simulink model "cov_compare"  (Simulink 5.0)
settings: Solver=ode45  StartTime=0.0  StopTime=10.0  RelTol=1e-3
values from neighbouring files (symbols this model uses):
  I = eye(3)    [build17StateSysDyn.m]    (also in build9StateSysDyn.m; cmigits28_model_01.mat = [1 0 0 0 0 0 0 0 0 0 0 0 ... (784 elements, 28x28)]; covupdate.m = eye(m))
undefined symbols (not defined in the file or in its folder): F1, F2, H1, H2, P1_0, P2_0, Q1, Q2, R1, R2, rss_ratio, ud_inv
libraries: simulink x4
settings Model: Creator=mcarroll  LastModifiedBy=mcarroll  ExtModeAutoUpdateStatusClock=off  SaveFormat=StructureWithTime

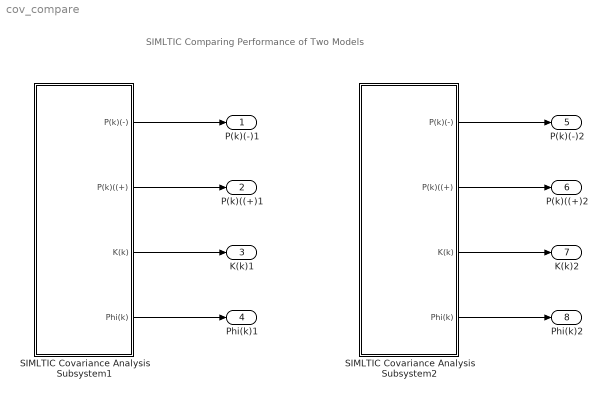
== system cov_compare ==
  note: SIMLTIC
      | Comparing Performance of Two Models
  SIMLTIC Covariance Analysis Subsystem1 : Subsystem
  SIMLTIC Covariance Analysis Subsystem2 : Subsystem
  P(k)(-)1 : Outport
  P(k)((+)1 : Outport  Port=2
  K(k)1 : Outport  Port=3
  Phi(k)1 : Outport  Port=4
  P(k)(-)2 : Outport  Port=5
  P(k)((+)2 : Outport  Port=6
  K(k)2 : Outport  Port=7
  Phi(k)2 : Outport  Port=8
  wires:
  SIMLTIC Covariance Analysis Subsystem1/1(P(k)(-)) -> P(k)(-)1/1
  SIMLTIC Covariance Analysis Subsystem1/2(P(k)((+)) -> P(k)((+)1/1
  SIMLTIC Covariance Analysis Subsystem1/3(K(k)) -> K(k)1/1
  SIMLTIC Covariance Analysis Subsystem1/4(Phi(k)) -> Phi(k)1/1
  SIMLTIC Covariance Analysis Subsystem2/1(P(k)(-)) -> P(k)(-)2/1
  SIMLTIC Covariance Analysis Subsystem2/2(P(k)((+)) -> P(k)((+)2/1
  SIMLTIC Covariance Analysis Subsystem2/3(K(k)) -> K(k)2/1
  SIMLTIC Covariance Analysis Subsystem2/4(Phi(k)) -> Phi(k)2/1

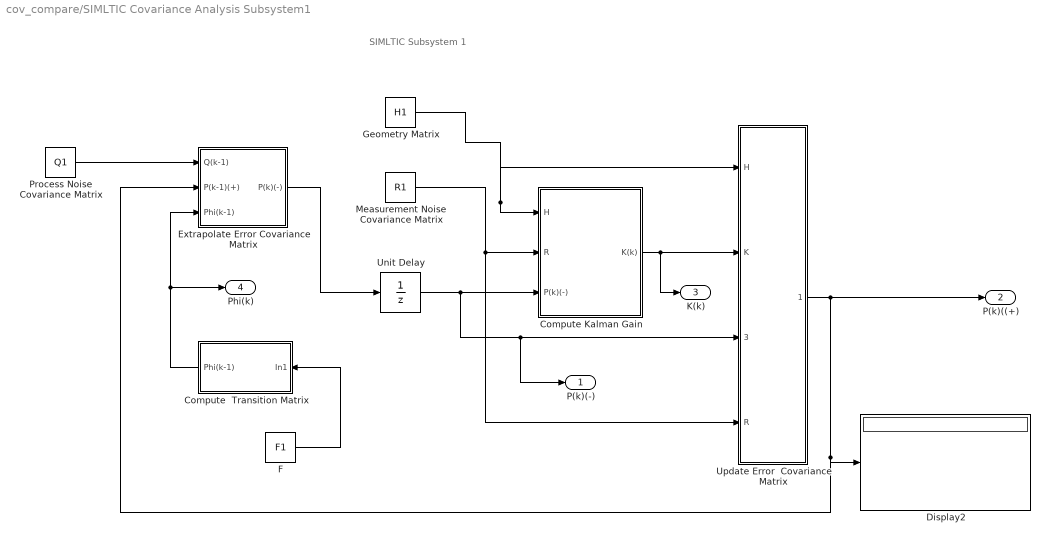
== system cov_compare/SIMLTIC Covariance Analysis Subsystem1 ==
  note: SIMLTIC
      | Subsystem 1
  Compute  Transition Matrix : Subsystem  Orientation=left
  Compute Kalman Gain : Subsystem
  Display2 : Display
  Extrapolate Error Covariance Matrix : Subsystem
  F : Constant  Value=F1  VectorParams1D=off
  Geometry Matrix : Constant  Value=H1  VectorParams1D=off
  Measurement Noise Covariance Matrix : Constant  Value=R1  VectorParams1D=off
  Process Noise Covariance Matrix : Constant  Value=Q1  VectorParams1D=off
  Unit Delay : UnitDelay  X0=P1_0
  Update Error  Covariance Matrix : Subsystem
  P(k)(-) : Outport
  P(k)((+) : Outport  Port=2
  K(k) : Outport  Port=3
  Phi(k) : Outport  Port=4
  wires:
  F/1 -> Compute  Transition Matrix/1(In1)
  Measurement Noise Covariance Matrix/1 -> Update Error  Covariance Matrix/4(R), Compute Kalman Gain/2(R)
  Geometry Matrix/1 -> Update Error  Covariance Matrix/1(H), Compute Kalman Gain/1(H)
  Compute  Transition Matrix/1(Phi(k-1)) -> Phi(k)/1, Extrapolate Error Covariance Matrix/3(Phi(k-1))
  Extrapolate Error Covariance Matrix/1(P(k)(-)) -> Unit Delay/1
  Process Noise Covariance Matrix/1 -> Extrapolate Error Covariance Matrix/1(Q(k-1))
  Compute Kalman Gain/1(K(k)) -> K(k)/1, Update Error  Covariance Matrix/2(K)
  Unit Delay/1 -> P(k)(-)/1, Update Error  Covariance Matrix/3(P(k)(-)), Compute Kalman Gain/3(P(k)(-))
  Update Error  Covariance Matrix/1(P(k)(+)) -> P(k)((+)/1, Extrapolate Error Covariance Matrix/2(P(k-1)(+)), Display2/1

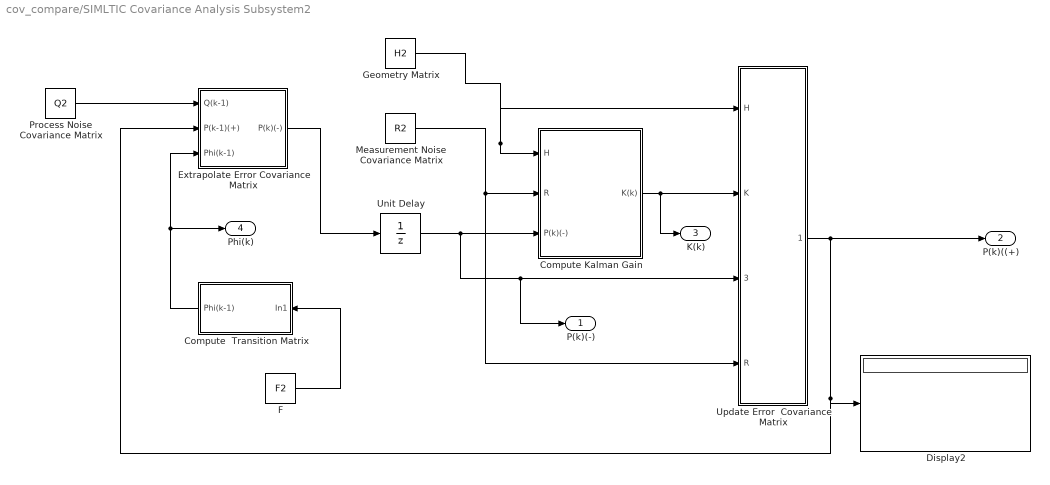
== system cov_compare/SIMLTIC Covariance Analysis Subsystem2 ==
  Compute  Transition Matrix : Subsystem  Orientation=left
  Compute Kalman Gain : Subsystem
  Display2 : Display
  Extrapolate Error Covariance Matrix : Subsystem
  F : Constant  Value=F2  VectorParams1D=off
  Geometry Matrix : Constant  Value=H2  VectorParams1D=off
  Measurement Noise Covariance Matrix : Constant  Value=R2  VectorParams1D=off
  Process Noise Covariance Matrix : Constant  Value=Q2  VectorParams1D=off
  Unit Delay : UnitDelay  X0=P2_0
  Update Error  Covariance Matrix : Subsystem
  P(k)(-) : Outport
  P(k)((+) : Outport  Port=2
  K(k) : Outport  Port=3
  Phi(k) : Outport  Port=4
  wires:
  Update Error  Covariance Matrix/1(P(k)(+)) -> Display2/1, Extrapolate Error Covariance Matrix/2(P(k-1)(+)), P(k)((+)/1
  Unit Delay/1 -> Compute Kalman Gain/3(P(k)(-)), Update Error  Covariance Matrix/3(P(k)(-)), P(k)(-)/1
  Compute Kalman Gain/1(K(k)) -> Update Error  Covariance Matrix/2(K), K(k)/1
  Process Noise Covariance Matrix/1 -> Extrapolate Error Covariance Matrix/1(Q(k-1))
  Extrapolate Error Covariance Matrix/1(P(k)(-)) -> Unit Delay/1
  Compute  Transition Matrix/1(Phi(k-1)) -> Extrapolate Error Covariance Matrix/3(Phi(k-1)), Phi(k)/1
  Geometry Matrix/1 -> Compute Kalman Gain/1(H), Update Error  Covariance Matrix/1(H)
  Measurement Noise Covariance Matrix/1 -> Compute Kalman Gain/2(R), Update Error  Covariance Matrix/4(R)
  F/1 -> Compute  Transition Matrix/1(In1)

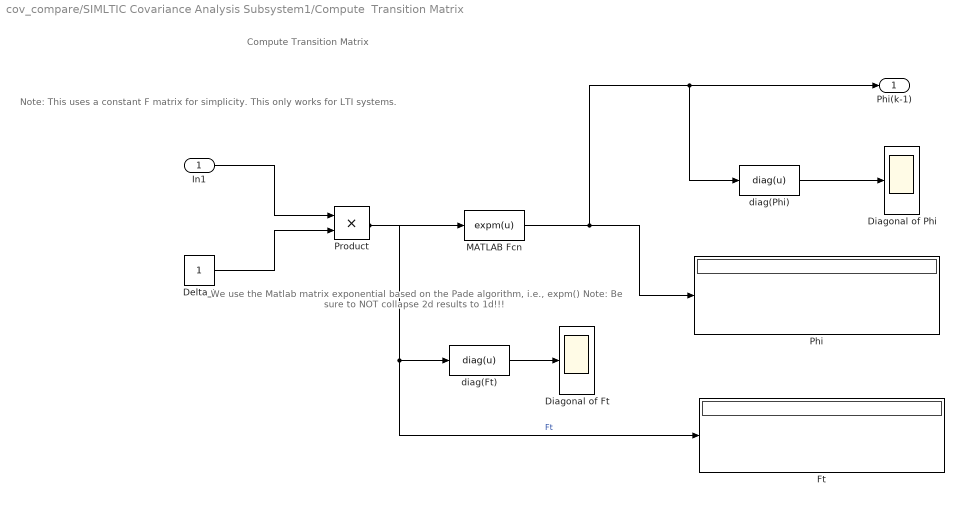
== system cov_compare/SIMLTIC Covariance Analysis Subsystem1/Compute  Transition Matrix ==
  note: Compute Transition Matrix
  note: Note:  This uses a constant F matrix
      | for simplicity.  This only works for LTI
      | systems.
  note: We use the Matlab matrix exponential based
      | on the Pade algorithm, i.e., expm()
      | Note:  Be sure to NOT collapse 2d results
      | to 1d!!!
  In1 : Inport
  Delta_t : Constant
  Diagonal of Ft : Scope
      settings: YMin=0  YMax=2  SaveName=ScopeData18
  Diagonal of Phi : Scope
      settings: YMin=0  YMax=2  SaveName=ScopeData3
  Ft : Display
  MATLAB Fcn : MATLABFcn  MATLABFcn=expm(u)  Output1D=off
  Phi : Display
  Product : Product  SaturateOnIntegerOverflow=on  InputSameDT=on
  diag(Ft) : MATLABFcn  MATLABFcn=diag(u)  Output1D=off
  diag(Phi) : MATLABFcn  MATLABFcn=diag(u)
  Phi(k-1) : Outport
  wires:
  In1/1 -> Product/1
  Product/1 -> MATLAB Fcn/1, Ft/1, diag(Ft)/1  "Ft"
  MATLAB Fcn/1 -> Phi/1, Phi(k-1)/1, diag(Phi)/1
  diag(Phi)/1 -> Diagonal of Phi/1
  diag(Ft)/1 -> Diagonal of Ft/1
  Delta_t/1 -> Product/2

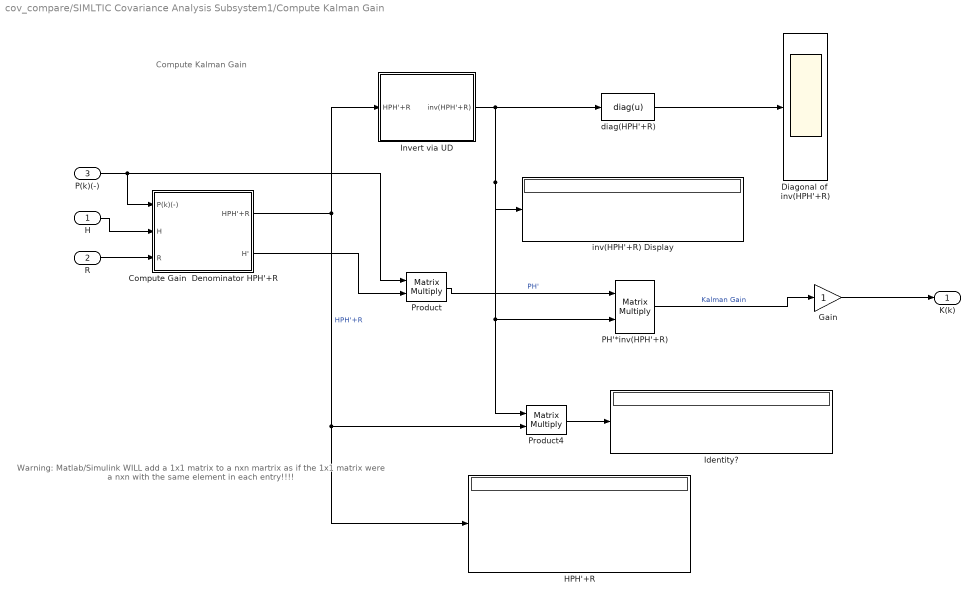
== system cov_compare/SIMLTIC Covariance Analysis Subsystem1/Compute Kalman Gain ==
  note: Warning:
      | Matlab/Simulink
      | WILL add a 1x1 matrix to
      | a nxn martrix as if the
      | 1x1 matrix were a
      | nxn with the same element
      | in each entry!!!!
  note: Compute Kalman Gain
  H : Inport
  R : Inport  Port=2
  P(k)(-) : Inport  Port=3  ShowAdditionalParam=on
  Compute Gain  Denominator HPH'+R : Subsystem
  Diagonal of  inv(HPH'+R) : Scope
      settings: TimeRange=100  YMin=0.0006  YMax=0.002  SaveName=ScopeData2
  Gain : Gain  SaturateOnIntegerOverflow=on
  HPH'+R : Display
  Identity? : Display
  Invert via UD : Subsystem
  PH'*inv(HPH'+R) : Product  Multiplication=Matrix(*)  ShowAdditionalParam=on
  Product : Product  Multiplication=Matrix(*)  SaturateOnIntegerOverflow=on
  Product4 : Product  Multiplication=Matrix(*)  ShowAdditionalParam=on  SaturateOnIntegerOverflow=on  InputSameDT=on
  diag(HPH'+R) : MATLABFcn  MATLABFcn=diag(u)
  inv(HPH'+R) Display : Display
  K(k) : Outport
  wires:
  Gain/1 -> K(k)/1
  PH'*inv(HPH'+R)/1 -> Gain/1  "Kalman Gain"
  P(k)(-)/1 -> Product/1, Compute Gain  Denominator HPH'+R/1(P(k)(-))
  H/1 -> Compute Gain  Denominator HPH'+R/2(H)
  Product4/1 -> Identity?/1
  Product/1 -> PH'*inv(HPH'+R)/1  "PH'"
  Compute Gain  Denominator HPH'+R/2(H') -> Product/2
  Invert via UD/1(inv(HPH'+R)) -> Product4/1, PH'*inv(HPH'+R)/2, inv(HPH'+R) Display/1, diag(HPH'+R)/1
  diag(HPH'+R)/1 -> Diagonal of  inv(HPH'+R)/1
  R/1 -> Compute Gain  Denominator HPH'+R/3(R)
  Compute Gain  Denominator HPH'+R/1(HPH'+R) -> Product4/2, HPH'+R/1, Invert via UD/1(HPH'+R)  "HPH'+R"

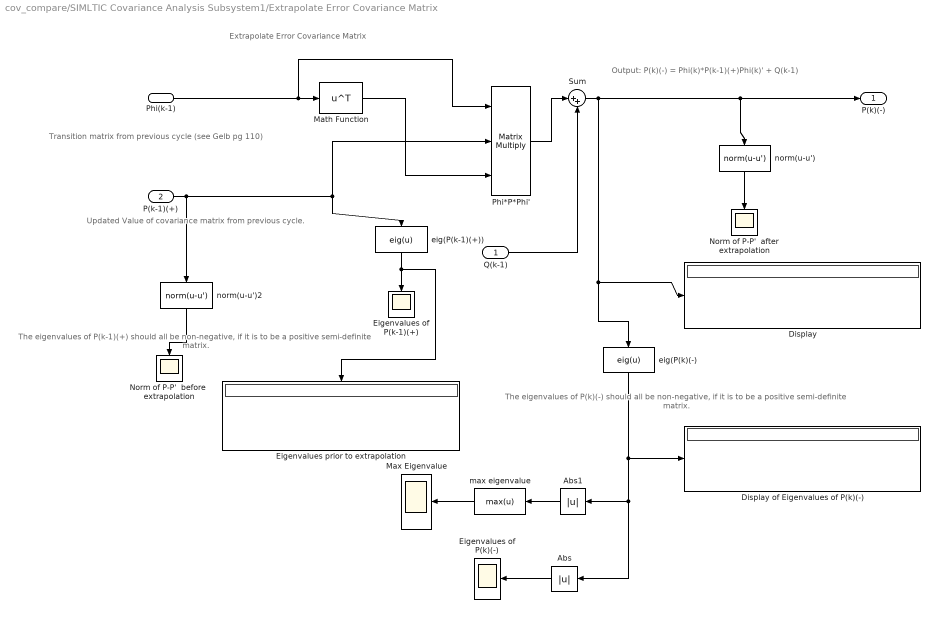
== system cov_compare/SIMLTIC Covariance Analysis Subsystem1/Extrapolate Error Covariance Matrix ==
  note: Extrapolate Error Covariance Matrix
  note: Updated Value of
      | covariance matrix  from
      | previous cycle.
  note: Output: P(k)(-) = Phi(k)*P(k-1)(+)Phi(k)' + Q(k-1)
  note: Transition matrix from
      | previous cycle
      | (see Gelb pg 110)
  note: The eigenvalues of P(k-1)(+) should all be
      | non-negative, if it is to be a positive
      | semi-definite matrix.
  note: The eigenvalues of P(k)(-) should all be non-negative,
      | if it is to be a positive semi-definite matrix.
  Q(k-1) : Inport
  P(k-1)(+) : Inport  Port=2
  Phi(k-1) : Inport  Port=3
  Abs : Abs  Orientation=left  SaturateOnIntegerOverflow=on
  Abs1 : Abs  Orientation=left  SaturateOnIntegerOverflow=on
  Display : Display
  Display of Eigenvalues of P(k)(-) : Display
  Eigenvalues prior to extrapolation : Display
      settings: Orientation=down
  Eigenvalues of P(k)(-) : Scope
      settings: SaveName=ScopeData8
  Eigenvalues of P(k-1)(+) : Scope
      settings: Orientation=down  YMin=1  YMax=8.5  SaveName=ScopeData7
  Math Function : Math  Operator=transpose
  Max Eigenvalue : Scope
      settings: TimeRange=100  YMin=0  YMax=4e+072  SaveName=ScopeData12
  Norm of P-P'  after extrapolation : Scope
      settings: Orientation=down  TimeRange=10  YMin=0  YMax=35  SaveName=ScopeData15
  Norm of P-P'  before  extrapolation : Scope
      settings: Orientation=down  TimeRange=10  YMin=0  YMax=35  SaveName=ScopeData16
  Phi*P*Phi' : Product  Inputs=3  Multiplication=Matrix(*)  SaturateOnIntegerOverflow=on  InputSameDT=on
  Sum : Sum  Inputs=|++  SaturateOnIntegerOverflow=on  InputSameDT=on
  eig(P(k)(-) : MATLABFcn  Orientation=down  MATLABFcn=eig(u)  OutputSignalType=complex
  eig(P(k-1)(+)) : MATLABFcn  Orientation=down  MATLABFcn=eig(u)
  max eigenvalue : MATLABFcn  Orientation=left  MATLABFcn=max(u)  Output1D=off
  norm(u-u') : MATLABFcn  Orientation=down  MATLABFcn=norm(u-u')  Output1D=off
  norm(u-u')2 : MATLABFcn  Orientation=down  MATLABFcn=norm(u-u')  Output1D=off
  P(k)(-) : Outport
  wires:
  Phi*P*Phi'/1 -> Sum/1
  Sum/1 -> Display/1, eig(P(k)(-)/1, P(k)(-)/1, norm(u-u')/1
  Phi(k-1)/1 -> Math Function/1, Phi*P*Phi'/1
  P(k-1)(+)/1 -> norm(u-u')2/1, eig(P(k-1)(+))/1, Phi*P*Phi'/2
  Q(k-1)/1 -> Sum/2
  eig(P(k-1)(+))/1 -> Eigenvalues of P(k-1)(+)/1, Eigenvalues prior to extrapolation/1
  eig(P(k)(-)/1 -> Display of Eigenvalues of P(k)(-)/1, Abs/1, Abs1/1
  norm(u-u')/1 -> Norm of P-P'  after extrapolation/1
  norm(u-u')2/1 -> Norm of P-P'  before  extrapolation/1
  Abs/1 -> Eigenvalues of P(k)(-)/1
  Abs1/1 -> max eigenvalue/1
  max eigenvalue/1 -> Max Eigenvalue/1
  Math Function/1 -> Phi*P*Phi'/3

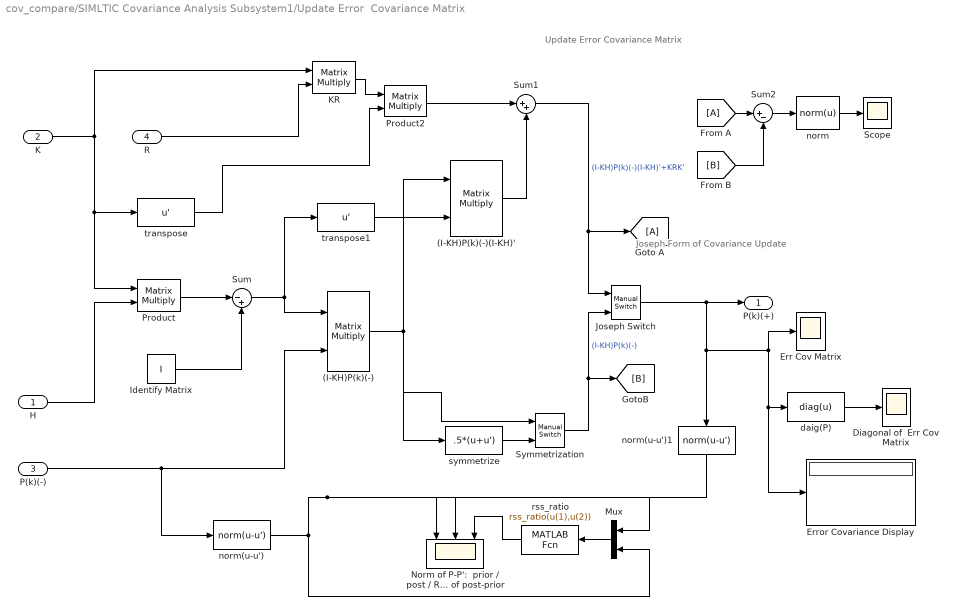
== system cov_compare/SIMLTIC Covariance Analysis Subsystem1/Update Error  Covariance Matrix ==
  note: Joseph Form
      | of Covariance
      | Update
  note: Update Error Covariance Matrix
  H : Inport
  K : Inport  Port=2  ShowAdditionalParam=on
  P(k)(-) : Inport  Port=3
  R : Inport  Port=4
  (I-KH)P(k)(-) : Product  Multiplication=Matrix(*)  SaturateOnIntegerOverflow=on  InputSameDT=on
  (I-KH)P(k)(-)(I-KH)' : Product  Multiplication=Matrix(*)  SaturateOnIntegerOverflow=on  InputSameDT=on
  Diagonal of  Err Cov Matrix : Scope
      settings: YMin=0  YMax=5000
  Err Cov Matrix : Scope
      settings: TimeRange=10  YMin=-60  YMax=80
  Error Covariance Display : Display
  Identify Matrix : Constant  Value=I  VectorParams1D=off
  Joseph Switch : simulink/Signal Routing/Manual Switch  sw=1  action=0
  KR : Product  Multiplication=Matrix(*)  SaturateOnIntegerOverflow=on
  Mux : Mux  Orientation=left  Inputs=2
  Norm of P-P':  prior / post / RSS ratio  of post-prior : Scope  NumInputPorts=3
      settings: Orientation=down  TimeRange=10  YMin=0~0~0  YMax=40~2~0.05  SaveName=ScopeData13
  Product : Product  Multiplication=Matrix(*)  SaturateOnIntegerOverflow=on  InputSameDT=on
  Product2 : Product  Multiplication=Matrix(*)  SaturateOnIntegerOverflow=on
  Scope : Scope
      settings: SaveName=ScopeData14
  Sum : Sum  Inputs=|-+  SaturateOnIntegerOverflow=on  InputSameDT=on
  Sum1 : Sum  Inputs=|++  SaturateOnIntegerOverflow=on  InputSameDT=on
  Sum2 : Sum  Inputs=|+-  SaturateOnIntegerOverflow=on  InputSameDT=on
  Symmetrization : simulink/Signal Routing/Manual Switch  sw=1  action=0
  daig(P) : MATLABFcn  MATLABFcn=diag(u)
  norm : MATLABFcn  MATLABFcn=norm(u)  Output1D=off
  norm(u-u') : MATLABFcn  MATLABFcn=norm(u-u')  Output1D=off
  norm(u-u')1 : MATLABFcn  Orientation=down  MATLABFcn=norm(u-u')  Output1D=off
  rss_ratio : MATLABFcn  Orientation=left  MATLABFcn=rss_ratio(u(1),u(2))  OutputSignalType=real
  symmetrize : MATLABFcn  MATLABFcn=.5*(u+u')  Output1D=off
  transpose : MATLABFcn  MATLABFcn=u'  Output1D=off
  transpose1 : MATLABFcn  MATLABFcn=u'  Output1D=off
  P(k)(+) : Outport
  wires:
  KR/1 -> Product2/1
  daig(P)/1 -> Diagonal of  Err Cov Matrix/1
  norm/1 -> Scope/1
  Sum2/1 -> norm/1
  [A] -> Sum2/1
  [B] -> Sum2/2
  Mux/1 -> rss_ratio/1
  rss_ratio/1 -> Norm of P-P':  prior / post / RSS ratio  of post-prior/3
  norm(u-u')1/1 -> Mux/1, Norm of P-P':  prior / post / RSS ratio  of post-prior/2
  norm(u-u')/1 -> Mux/2, Norm of P-P':  prior / post / RSS ratio  of post-prior/1
  Sum1/1 -> [A], Joseph Switch/1  "(I-KH)P(k)(-)(I-KH)'+KRK'"
  Joseph Switch/1 -> Err Cov Matrix/1, Error Covariance Display/1, daig(P)/1, norm(u-u')1/1, P(k)(+)/1
  Symmetrization/1 -> [B], Joseph Switch/2  "(I-KH)P(k)(-)"
  symmetrize/1 -> Symmetrization/2
  Product2/1 -> Sum1/1
  (I-KH)P(k)(-)(I-KH)'/1 -> Sum1/2
  transpose1/1 -> (I-KH)P(k)(-)(I-KH)'/2
  (I-KH)P(k)(-)/1 -> symmetrize/1, Symmetrization/1, (I-KH)P(k)(-)(I-KH)'/1
  transpose/1 -> Product2/2
  R/1 -> KR/2
  Sum/1 -> transpose1/1, (I-KH)P(k)(-)/1
  Product/1 -> Sum/1
  Identify Matrix/1 -> Sum/2
  P(k)(-)/1 -> norm(u-u')/1, (I-KH)P(k)(-)/2
  K/1 -> KR/1, transpose/1, Product/1
  H/1 -> Product/2

== system cov_compare/SIMLTIC Covariance Analysis Subsystem2/Compute  Transition Matrix ==
  note: We use the Matlab matrix exponential based
      | on the Pade algorithm, i.e., expm()
      | Note:  Be sure to NOT collapse 2d results
      | to 1d!!!
  note: Note:  This uses a constant F matrix
      | for simplicity.  This only works for LTI
      | systems.
  note: Compute Transition Matrix
  In1 : Inport
  Delta_t : Constant
  Diagonal of Ft : Scope
      settings: YMin=0  YMax=2  SaveName=ScopeData18
  Diagonal of Phi : Scope
      settings: YMin=0  YMax=2  SaveName=ScopeData3
  Ft : Display
  MATLAB Fcn : MATLABFcn  MATLABFcn=expm(u)  Output1D=off
  Phi : Display
  Product : Product  SaturateOnIntegerOverflow=on  InputSameDT=on
  diag(Ft) : MATLABFcn  MATLABFcn=diag(u)  Output1D=off
  diag(Phi) : MATLABFcn  MATLABFcn=diag(u)
  Phi(k-1) : Outport
  wires:
  Delta_t/1 -> Product/2
  diag(Ft)/1 -> Diagonal of Ft/1
  diag(Phi)/1 -> Diagonal of Phi/1
  MATLAB Fcn/1 -> diag(Phi)/1, Phi(k-1)/1, Phi/1
  Product/1 -> diag(Ft)/1, Ft/1, MATLAB Fcn/1  "Ft"
  In1/1 -> Product/1

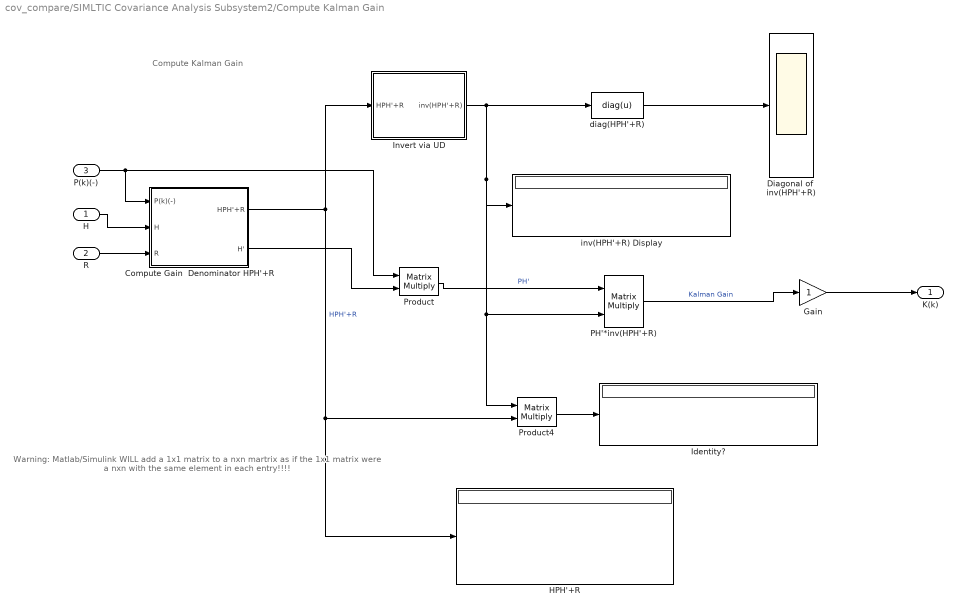
== system cov_compare/SIMLTIC Covariance Analysis Subsystem2/Compute Kalman Gain ==
  note: Compute Kalman Gain
  note: Warning:
      | Matlab/Simulink
      | WILL add a 1x1 matrix to
      | a nxn martrix as if the
      | 1x1 matrix were a
      | nxn with the same element
      | in each entry!!!!
  H : Inport
  R : Inport  Port=2
  P(k)(-) : Inport  Port=3  ShowAdditionalParam=on
  Compute Gain  Denominator HPH'+R : Subsystem
  Diagonal of  inv(HPH'+R) : Scope
      settings: TimeRange=100  YMin=0.0006  YMax=0.002  SaveName=ScopeData2
  Gain : Gain  SaturateOnIntegerOverflow=on
  HPH'+R : Display
  Identity? : Display
  Invert via UD : Subsystem
  PH'*inv(HPH'+R) : Product  Multiplication=Matrix(*)  ShowAdditionalParam=on
  Product : Product  Multiplication=Matrix(*)  SaturateOnIntegerOverflow=on
  Product4 : Product  Multiplication=Matrix(*)  ShowAdditionalParam=on  SaturateOnIntegerOverflow=on  InputSameDT=on
  diag(HPH'+R) : MATLABFcn  MATLABFcn=diag(u)
  inv(HPH'+R) Display : Display
  K(k) : Outport
  wires:
  Compute Gain  Denominator HPH'+R/1(HPH'+R) -> Invert via UD/1(HPH'+R), HPH'+R/1, Product4/2  "HPH'+R"
  R/1 -> Compute Gain  Denominator HPH'+R/3(R)
  diag(HPH'+R)/1 -> Diagonal of  inv(HPH'+R)/1
  Invert via UD/1(inv(HPH'+R)) -> diag(HPH'+R)/1, inv(HPH'+R) Display/1, PH'*inv(HPH'+R)/2, Product4/1
  Compute Gain  Denominator HPH'+R/2(H') -> Product/2
  Product/1 -> PH'*inv(HPH'+R)/1  "PH'"
  Product4/1 -> Identity?/1
  H/1 -> Compute Gain  Denominator HPH'+R/2(H)
  P(k)(-)/1 -> Compute Gain  Denominator HPH'+R/1(P(k)(-)), Product/1
  PH'*inv(HPH'+R)/1 -> Gain/1  "Kalman Gain"
  Gain/1 -> K(k)/1

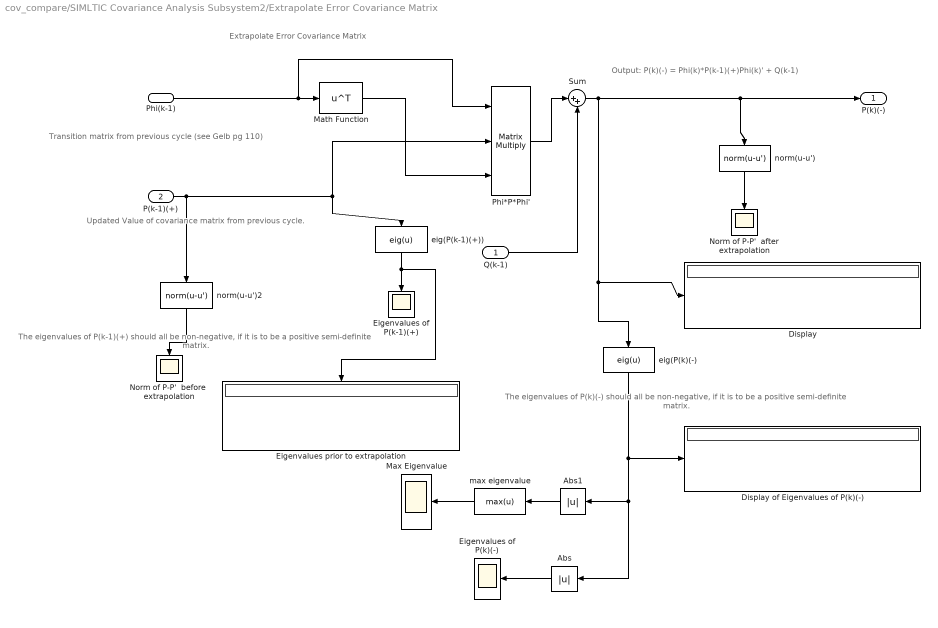
== system cov_compare/SIMLTIC Covariance Analysis Subsystem2/Extrapolate Error Covariance Matrix ==
  note: The eigenvalues of P(k)(-) should all be non-negative,
      | if it is to be a positive semi-definite matrix.
  note: The eigenvalues of P(k-1)(+) should all be
      | non-negative, if it is to be a positive
      | semi-definite matrix.
  note: Transition matrix from
      | previous cycle
      | (see Gelb pg 110)
  note: Output: P(k)(-) = Phi(k)*P(k-1)(+)Phi(k)' + Q(k-1)
  note: Updated Value of
      | covariance matrix  from
      | previous cycle.
  note: Extrapolate Error Covariance Matrix
  Q(k-1) : Inport
  P(k-1)(+) : Inport  Port=2
  Phi(k-1) : Inport  Port=3
  Abs : Abs  Orientation=left  SaturateOnIntegerOverflow=on
  Abs1 : Abs  Orientation=left  SaturateOnIntegerOverflow=on
  Display : Display
  Display of Eigenvalues of P(k)(-) : Display
  Eigenvalues prior to extrapolation : Display
      settings: Orientation=down
  Eigenvalues of P(k)(-) : Scope
      settings: SaveName=ScopeData8
  Eigenvalues of P(k-1)(+) : Scope
      settings: Orientation=down  YMin=1  YMax=8.5  SaveName=ScopeData7
  Math Function : Math  Operator=transpose
  Max Eigenvalue : Scope
      settings: TimeRange=100  YMin=0  YMax=4e+072  SaveName=ScopeData12
  Norm of P-P'  after extrapolation : Scope
      settings: Orientation=down  TimeRange=10  YMin=0  YMax=35  SaveName=ScopeData15
  Norm of P-P'  before  extrapolation : Scope
      settings: Orientation=down  TimeRange=10  YMin=0  YMax=35  SaveName=ScopeData16
  Phi*P*Phi' : Product  Inputs=3  Multiplication=Matrix(*)  SaturateOnIntegerOverflow=on  InputSameDT=on
  Sum : Sum  Inputs=|++  SaturateOnIntegerOverflow=on  InputSameDT=on
  eig(P(k)(-) : MATLABFcn  Orientation=down  MATLABFcn=eig(u)  OutputSignalType=complex
  eig(P(k-1)(+)) : MATLABFcn  Orientation=down  MATLABFcn=eig(u)
  max eigenvalue : MATLABFcn  Orientation=left  MATLABFcn=max(u)  Output1D=off
  norm(u-u') : MATLABFcn  Orientation=down  MATLABFcn=norm(u-u')  Output1D=off
  norm(u-u')2 : MATLABFcn  Orientation=down  MATLABFcn=norm(u-u')  Output1D=off
  P(k)(-) : Outport
  wires:
  Math Function/1 -> Phi*P*Phi'/3
  max eigenvalue/1 -> Max Eigenvalue/1
  Abs1/1 -> max eigenvalue/1
  Abs/1 -> Eigenvalues of P(k)(-)/1
  norm(u-u')2/1 -> Norm of P-P'  before  extrapolation/1
  norm(u-u')/1 -> Norm of P-P'  after extrapolation/1
  eig(P(k)(-)/1 -> Abs1/1, Abs/1, Display of Eigenvalues of P(k)(-)/1
  eig(P(k-1)(+))/1 -> Eigenvalues prior to extrapolation/1, Eigenvalues of P(k-1)(+)/1
  Q(k-1)/1 -> Sum/2
  P(k-1)(+)/1 -> Phi*P*Phi'/2, eig(P(k-1)(+))/1, norm(u-u')2/1
  Phi(k-1)/1 -> Phi*P*Phi'/1, Math Function/1
  Sum/1 -> norm(u-u')/1, P(k)(-)/1, eig(P(k)(-)/1, Display/1
  Phi*P*Phi'/1 -> Sum/1

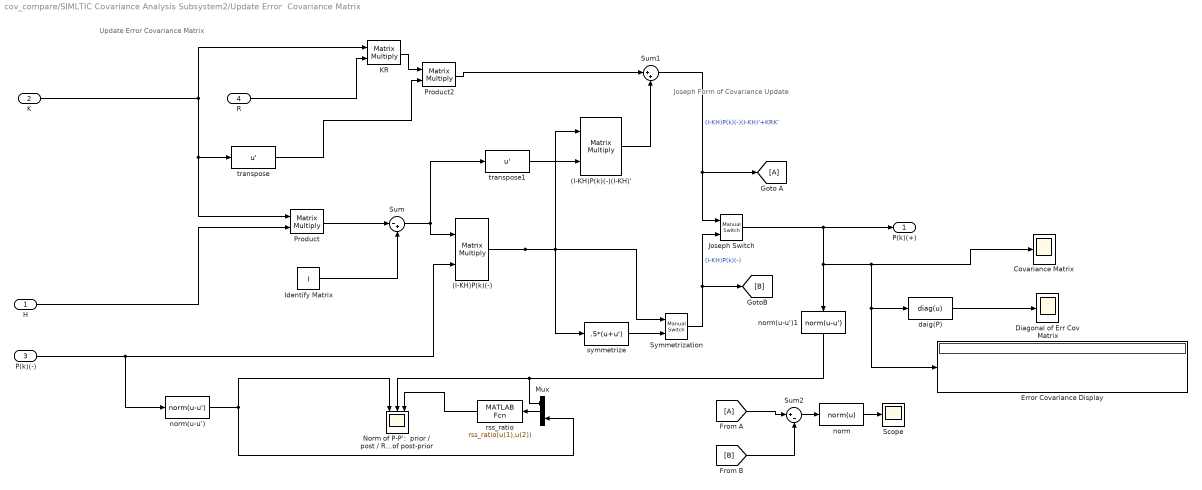
== system cov_compare/SIMLTIC Covariance Analysis Subsystem2/Update Error  Covariance Matrix ==
  note: Update Error Covariance Matrix
  note: Joseph Form
      | of Covariance
      | Update
  H : Inport
  K : Inport  Port=2  ShowAdditionalParam=on
  P(k)(-) : Inport  Port=3
  R : Inport  Port=4
  (I-KH)P(k)(-) : Product  Multiplication=Matrix(*)  SaturateOnIntegerOverflow=on  InputSameDT=on
  (I-KH)P(k)(-)(I-KH)' : Product  Multiplication=Matrix(*)  SaturateOnIntegerOverflow=on  InputSameDT=on
  Covariance Matrix : Scope
      settings: TimeRange=10  YMin=-60  YMax=80
  Diagonal of Err Cov Matrix : Scope
      settings: YMin=0  YMax=5000
  Error Covariance Display : Display
  Identify Matrix : Constant  Value=I  VectorParams1D=off
  Joseph Switch : simulink/Signal Routing/Manual Switch  sw=1  action=0
  KR : Product  Multiplication=Matrix(*)  SaturateOnIntegerOverflow=on
  Mux : Mux  Orientation=left  Inputs=2
  Norm of P-P':  prior / post / RSS ratio of post-prior : Scope  NumInputPorts=3
      settings: Orientation=down  TimeRange=10  YMin=0~0~0  YMax=40~2~0.05  SaveName=ScopeData13
  Product : Product  Multiplication=Matrix(*)  SaturateOnIntegerOverflow=on  InputSameDT=on
  Product2 : Product  Multiplication=Matrix(*)  SaturateOnIntegerOverflow=on
  Scope : Scope
      settings: SaveName=ScopeData14
  Sum : Sum  Inputs=|-+  SaturateOnIntegerOverflow=on  InputSameDT=on
  Sum1 : Sum  Inputs=|++  SaturateOnIntegerOverflow=on  InputSameDT=on
  Sum2 : Sum  Inputs=|+-  SaturateOnIntegerOverflow=on  InputSameDT=on
  Symmetrization : simulink/Signal Routing/Manual Switch  sw=1  action=0
  daig(P) : MATLABFcn  MATLABFcn=diag(u)
  norm : MATLABFcn  MATLABFcn=norm(u)  Output1D=off
  norm(u-u') : MATLABFcn  MATLABFcn=norm(u-u')  Output1D=off
  norm(u-u')1 : MATLABFcn  Orientation=down  MATLABFcn=norm(u-u')  Output1D=off
  rss_ratio : MATLABFcn  Orientation=left  MATLABFcn=rss_ratio(u(1),u(2))  OutputSignalType=real
  symmetrize : MATLABFcn  MATLABFcn=.5*(u+u')  Output1D=off
  transpose : MATLABFcn  MATLABFcn=u'  Output1D=off
  transpose1 : MATLABFcn  MATLABFcn=u'  Output1D=off
  P(k)(+) : Outport
  wires:
  H/1 -> Product/2
  K/1 -> Product/1, transpose/1, KR/1
  P(k)(-)/1 -> (I-KH)P(k)(-)/2, norm(u-u')/1
  Identify Matrix/1 -> Sum/2
  Product/1 -> Sum/1
  Sum/1 -> (I-KH)P(k)(-)/1, transpose1/1
  R/1 -> KR/2
  transpose/1 -> Product2/2
  (I-KH)P(k)(-)/1 -> (I-KH)P(k)(-)(I-KH)'/1, Symmetrization/1, symmetrize/1
  transpose1/1 -> (I-KH)P(k)(-)(I-KH)'/2
  (I-KH)P(k)(-)(I-KH)'/1 -> Sum1/2
  Product2/1 -> Sum1/1
  symmetrize/1 -> Symmetrization/2
  Symmetrization/1 -> Joseph Switch/2, [B]  "(I-KH)P(k)(-)"
  Joseph Switch/1 -> P(k)(+)/1, norm(u-u')1/1, daig(P)/1, Error Covariance Display/1, Covariance Matrix/1
  Sum1/1 -> Joseph Switch/1, [A]  "(I-KH)P(k)(-)(I-KH)'+KRK'"
  norm(u-u')/1 -> Norm of P-P':  prior / post / RSS ratio of post-prior/1, Mux/2
  norm(u-u')1/1 -> Norm of P-P':  prior / post / RSS ratio of post-prior/2, Mux/1
  rss_ratio/1 -> Norm of P-P':  prior / post / RSS ratio of post-prior/3
  Mux/1 -> rss_ratio/1
  [B] -> Sum2/2
  [A] -> Sum2/1
  Sum2/1 -> norm/1
  norm/1 -> Scope/1
  daig(P)/1 -> Diagonal of Err Cov Matrix/1
  KR/1 -> Product2/1

== system cov_compare/SIMLTIC Covariance Analysis Subsystem1/Compute Kalman Gain/Compute Gain  Denominator HPH'+R ==
  note: Compute Gain Denominator
  P(k)(-) : Inport
  H : Inport  Port=2
  R : Inport  Port=3
  Product : Product  Multiplication=Matrix(*)  SaturateOnIntegerOverflow=on  InputSameDT=on
  Product1 : Product  Multiplication=Matrix(*)  ShowAdditionalParam=on  SaturateOnIntegerOverflow=on  InputSameDT=on
  Sum : Sum  Inputs=|++  SaturateOnIntegerOverflow=on  InputSameDT=on
  transpose : Math  Operator=transpose
  HPH'+R : Outport
  H' : Outport  Port=2
  wires:
  P(k)(-)/1 -> Product/2
  Sum/1 -> HPH'+R/1
  R/1 -> Sum/1
  H/1 -> transpose/1, Product/1
  Product/1 -> Product1/1  "HP"
  Product1/1 -> Sum/2  "HPH'"
  transpose/1 -> Product1/2, H'/1  "H'"

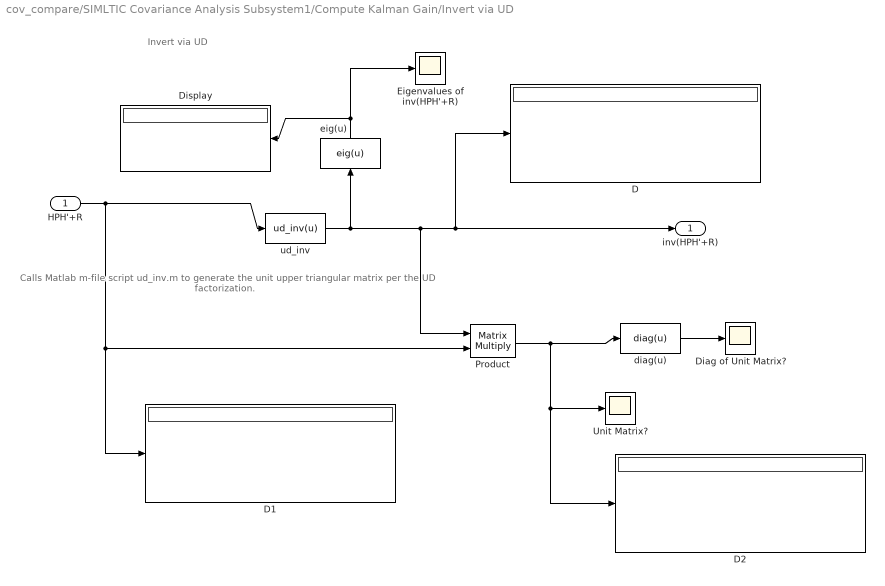
== system cov_compare/SIMLTIC Covariance Analysis Subsystem1/Compute Kalman Gain/Invert via UD ==
  note: Invert via UD
  note: Calls Matlab m-file script ud_inv.m
      | to generate the unit upper triangular
      | matrix per the UD factorization.
  HPH'+R : Inport
  D : Display
  D1 : Display
  D2 : Display
  Diag of Unit Matrix? : Scope
      settings: YMin=0.99  YMax=1.03  SaveName=ScopeData10
  Display : Display
  Eigenvalues of inv(HPH'+R) : Scope
      settings: SaveName=ScopeData6
  Product : Product  Multiplication=Matrix(*)  SaturateOnIntegerOverflow=on  InputSameDT=on
  Unit Matrix? : Scope
      settings: SaveName=ScopeData9
  diag(u) : MATLABFcn  MATLABFcn=diag(u)  Output1D=off
  eig(u) : MATLABFcn  Orientation=up  MATLABFcn=eig(u)  Output1D=off
  ud_inv : MATLABFcn  MATLABFcn=ud_inv(u)  Output1D=off
  inv(HPH'+R) : Outport
  wires:
  diag(u)/1 -> Diag of Unit Matrix?/1
  Product/1 -> D2/1, Unit Matrix?/1, diag(u)/1
  eig(u)/1 -> Display/1, Eigenvalues of inv(HPH'+R)/1
  ud_inv/1 -> Product/1, D/1, inv(HPH'+R)/1, eig(u)/1
  HPH'+R/1 -> Product/2, D1/1, ud_inv/1

== system cov_compare/SIMLTIC Covariance Analysis Subsystem2/Compute Kalman Gain/Compute Gain  Denominator HPH'+R ==
  note: Compute Gain Denominator
  P(k)(-) : Inport
  H : Inport  Port=2
  R : Inport  Port=3
  Product : Product  Multiplication=Matrix(*)  SaturateOnIntegerOverflow=on  InputSameDT=on
  Product1 : Product  Multiplication=Matrix(*)  ShowAdditionalParam=on  SaturateOnIntegerOverflow=on  InputSameDT=on
  Sum : Sum  Inputs=|++  SaturateOnIntegerOverflow=on  InputSameDT=on
  transpose : Math  Operator=transpose
  HPH'+R : Outport
  H' : Outport  Port=2
  wires:
  transpose/1 -> H'/1, Product1/2  "H'"
  Product1/1 -> Sum/2  "HPH'"
  Product/1 -> Product1/1  "HP"
  H/1 -> Product/1, transpose/1
  R/1 -> Sum/1
  Sum/1 -> HPH'+R/1
  P(k)(-)/1 -> Product/2

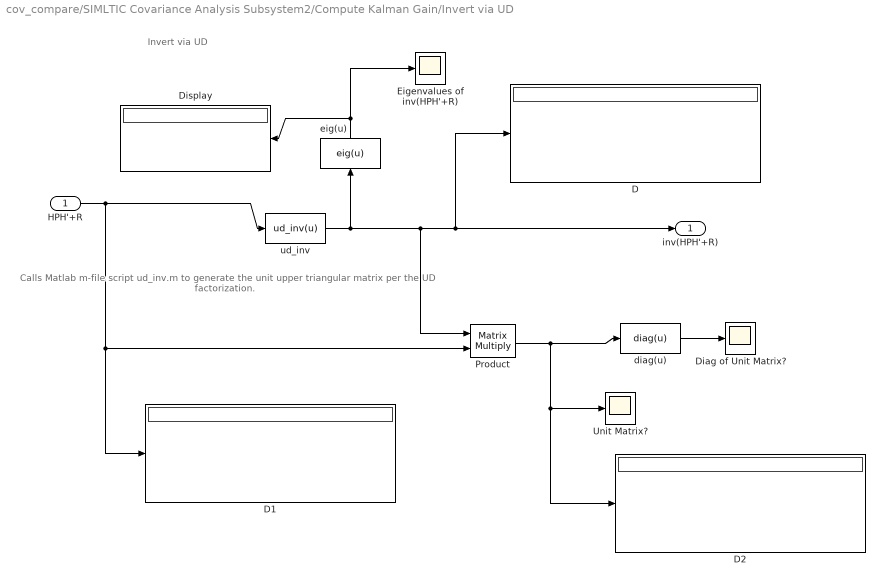
== system cov_compare/SIMLTIC Covariance Analysis Subsystem2/Compute Kalman Gain/Invert via UD ==
  note: Calls Matlab m-file script ud_inv.m
      | to generate the unit upper triangular
      | matrix per the UD factorization.
  note: Invert via UD
  HPH'+R : Inport
  D : Display
  D1 : Display
  D2 : Display
  Diag of Unit Matrix? : Scope
      settings: YMin=0.99  YMax=1.03  SaveName=ScopeData10
  Display : Display
  Eigenvalues of inv(HPH'+R) : Scope
      settings: SaveName=ScopeData6
  Product : Product  Multiplication=Matrix(*)  SaturateOnIntegerOverflow=on  InputSameDT=on
  Unit Matrix? : Scope
      settings: SaveName=ScopeData9
  diag(u) : MATLABFcn  MATLABFcn=diag(u)  Output1D=off
  eig(u) : MATLABFcn  Orientation=up  MATLABFcn=eig(u)  Output1D=off
  ud_inv : MATLABFcn  MATLABFcn=ud_inv(u)  Output1D=off
  inv(HPH'+R) : Outport
  wires:
  HPH'+R/1 -> ud_inv/1, D1/1, Product/2
  ud_inv/1 -> eig(u)/1, inv(HPH'+R)/1, D/1, Product/1
  eig(u)/1 -> Eigenvalues of inv(HPH'+R)/1, Display/1
  Product/1 -> diag(u)/1, Unit Matrix?/1, D2/1
  diag(u)/1 -> Diag of Unit Matrix?/1
